simulink model "BINS"  (Simulink 8.3)
settings: Solver=ode45  StartTime=0.0  StopTime=10.0  RelTol=1e-3
settings Model: Creator=me  LastModifiedBy=me
settings DataIOCC: SignalLoggingSaveFormat=Dataset
settings DebuggingCC: UnderspecifiedInitializationDetection=Simplified  StateNameClashWarn=none
settings GRTTargetCC: CombineOutputUpdateFcns=on  GRTInterface=off

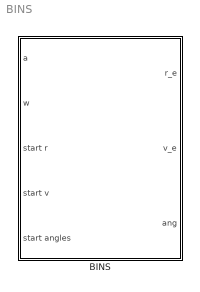
== system BINS ==
  BINS : Subsystem

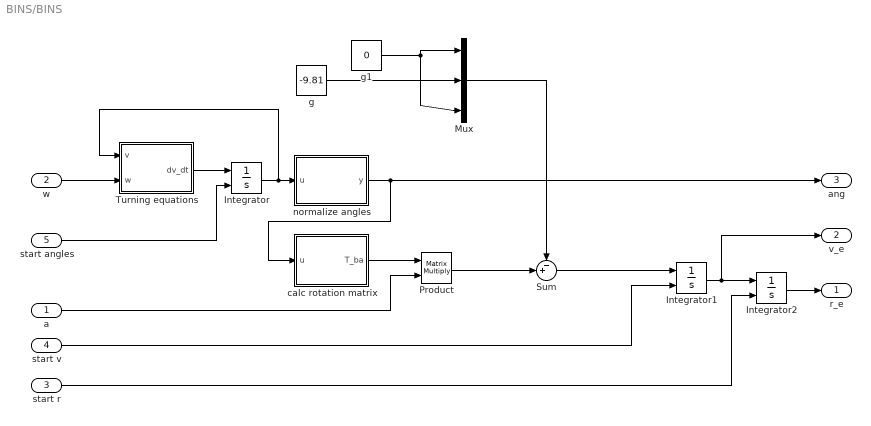
== system BINS/BINS ==
  a : Inport
  "w " : Inport  Port=2
  start r : Inport  Port=3
  start v : Inport  Port=4
  start angles : Inport  Port=5
  Integrator : Integrator  InitialConditionSource=external
  Integrator1 : Integrator  InitialConditionSource=external
  Integrator2 : Integrator  InitialConditionSource=external
  Mux : Mux  Inputs=3
  Product : Product  Multiplication=Matrix(*)
  Sum : Sum  Inputs=-+|
  Turning equations : MATLAB Function  TreatAsAtomicUnit=on
  calc rotation matrix : MATLAB Function  TreatAsAtomicUnit=on
  g : Constant  Value=-9.81
  g1 : Constant  Value=0
  normalize angles : MATLAB Function  TreatAsAtomicUnit=on
  r_e : Outport
  v_e : Outport  Port=2
  ang : Outport  Port=3
  wires:
  Turning equations/1(dv_dt) -> Integrator/1
  Integrator/1 -> Turning equations/1(v), normalize angles/1(u)
  normalize angles/1(y) -> calc rotation matrix/1(u), ang/1
  Integrator1/1 -> Integrator2/1, v_e/1
  start r/1 -> Integrator2/2
  a/1 -> Product/2
  start v/1 -> Integrator1/2
  start angles/1 -> Integrator/2
  calc rotation matrix/1(T_ba) -> Product/1
  Integrator2/1 -> r_e/1
  "w "/1 -> Turning equations/2(w)
  Product/1 -> Sum/2
  Sum/1 -> Integrator1/1
  g/1 -> Mux/2
  g1/1 -> Mux/3, Mux/1
  Mux/1 -> Sum/1

== matlab function BINS/Turning equations ==
  data: v input double; dv_dt output double; w input double
function dv_dt = fcn(v, w)
%#codegen

    dv_dt = f_turning_by_Euler(v, w);
    
end

== matlab function BINS/normalize angles ==
  data: u input double; y output double
function y = fcn(u)
%#codegen
y = u;
for i=1:length(y)
    y(i)=f_normalize_angle(u(i));
end

== matlab function BINS/calc rotation matrix ==
  data: u input double; T_ba output double
function T_ba = fcn(u)
%#codegen

T_ba = f_calc_turn_matrix_from_angles(u);
